simulink model "uavStepResponse"  (R2021b)
settings: configuration reference "ctrlConfigSet" (kept outside this file)
values from neighbouring files (symbols this model uses):
  TFinal = 200.0    [uavStepResponseData.sldd]
libraries: uavalgslib x1
settings Model: DataDictionary=uavStepResponseData.sldd  EnableAccessToBaseWorkspace=off  SimulationMode=accelerator  Creator=The MathWorks, Inc.  LastModifiedBy=The MathWorks, Inc.
settings ConfigSetRef: SourceName=ctrlConfigSet

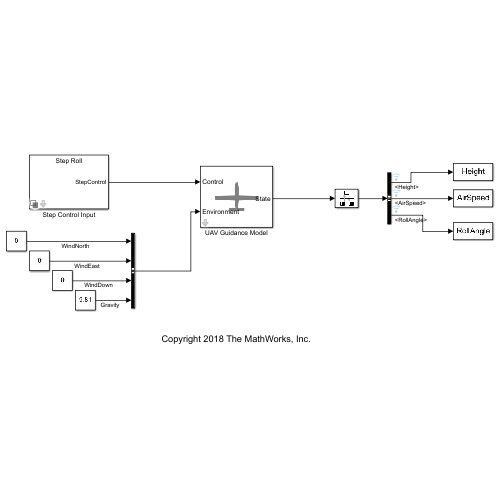
[thumbnail: Simulink's stored preview of the top-level diagram]
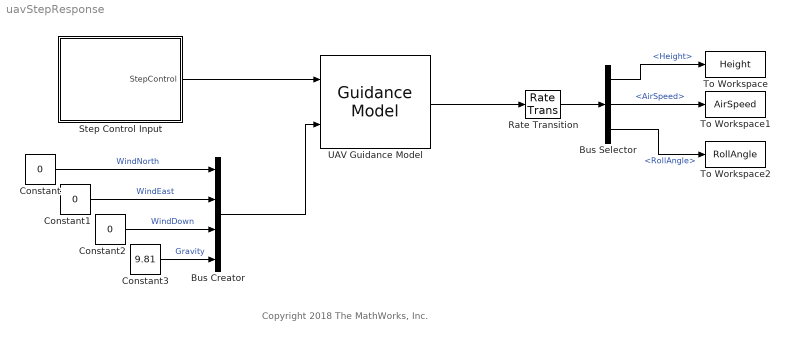
== system uavStepResponse ==
  note: Copyright 2018 The MathWorks, Inc.
  Bus Creator : BusCreator  Inputs=4  OutDataTypeStr=Bus: FixedWingEnvironmentBus  NonVirtualBus=on
  Bus Selector : BusSelector  OutputSignals=Height,AirSpeed,RollAngle
  Constant : Constant  Value=0
  Constant1 : Constant  Value=0
  Constant2 : Constant  Value=0
  Constant3 : Constant  Value=9.81
  Rate Transition : RateTransition  OutPortSampleTime=0.1
  Step Control Input : Subsystem  Variant=on  VariantControlMode=label  LabelModeActiveChoice=StepRollAngle  mask{StepControl=RollAngle Step Control}
      mask prompts: StepControl "Step control mode:"
      mask init:
      | switch StepControl
      |     case 1
      |         set_param(gcb,'LabelModeActiveChoice', 'StepHeight');
      |     case 2
      |         set_param(gcb,'LabelModeActiveChoice', 'StepAirSpeed');
      |     case 3
      |         set_param(gcb,'LabelModeActiveChoice', 'StepRollAngle');
      | end
      mask TypeOptions StepControl: Height Step Control | AirSpeed Step Control | RollAngle Step Control
  To Workspace : ToWorkspace  VariableName=Height  SaveFormat=Timeseries  SampleTime=-1
  To Workspace1 : ToWorkspace  VariableName=AirSpeed  SaveFormat=Timeseries  SampleTime=-1
  To Workspace2 : ToWorkspace  VariableName=RollAngle  SaveFormat=Timeseries  SampleTime=-1
  UAV Guidance Model : uavalgslib/Guidance Model  ModelType=FixedWingGuidance  SpecifiedDataType=double  SimulateUsing=Code generation  InitialWorldPositionMultirotor=[0; 0; 0]  InitialWorldVelocityMultirotor=[0; 0; 0]  InitialEulerZYXMultirotor=[0; 0; 0]  InitialBodyAngularRateRPYMultirotor=[0; 0; 0]  InitialThrustMultirotor=0  InitialNorthFixedWing=0  InitialEastFixedWing=0  InitialHeightFixedWing=0  InitialAirSpeedFixedWing=15  InitialHeadingAngleFixedWing=0  InitialFlightPathAngleFixedWing=0  InitialRollAngleFixedWing=0  InitialRollAngleRateFixedWing=0  PDRollMultirotor=[3402.97,116.67]  PDPitchMultirotor=[3402.97, 116.67]  PYawRateMultirotor=1950  PThrustMultirotor=3900  MassMultirotor=0.1  PHeightFixedWing=3.9  PHeadingAngleFixedWing=3.9  PFlightPathAngleFixedWing=39  PDRollFixedWing=[5.9414, 3.9]  PAirSpeedFixedWing=1  FlightPathAngleLimitsFixedWing=[-pi/6, pi/6]  StateBusName='FixedWingStateBus'  ControlBusName='FixedWingControlBus'  EnvironmentBusName='FixedWingEnvironmentBus'  DataType=double
      settings: SourceProductBaseCode=UV
  wires:
  Bus Selector/1 -> To Workspace/1  "<Height>"
  Bus Selector/2 -> To Workspace1/1  "<AirSpeed>"
  Bus Selector/3 -> To Workspace2/1  "<RollAngle>"
  Step Control Input/1(StepControl) -> UAV Guidance Model/1
  UAV Guidance Model/1 -> Rate Transition/1
  Rate Transition/1 -> Bus Selector/1
  Bus Creator/1 -> UAV Guidance Model/2
  Constant/1 -> Bus Creator/1  "WindNorth"
  Constant1/1 -> Bus Creator/2  "WindEast"
  Constant2/1 -> Bus Creator/3  "WindDown"
  Constant3/1 -> Bus Creator/4  "Gravity"

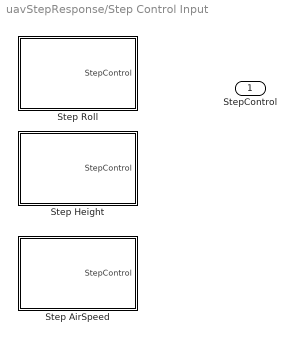
== system uavStepResponse/Step Control Input ==
  Step AirSpeed : Subsystem  VariantControl=StepAirSpeed
  Step Height : Subsystem  VariantControl=StepHeight
  Step Roll : Subsystem  VariantControl=StepRollAngle
  StepControl : Outport  VectorParamsAs1DForOutWhenUnconnected=off

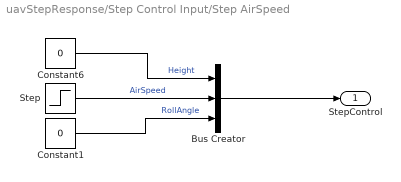
== system uavStepResponse/Step Control Input/Step AirSpeed ==
  Bus Creator : BusCreator  Inputs=3  OutDataTypeStr=Bus: FixedWingControlBus  NonVirtualBus=on
  Constant1 : Constant  Value=0
  Constant6 : Constant  Value=0
  Step : Step  Time=TFinal/2  Before=15  After=16  SampleTime=0
  StepControl : Outport  VectorParamsAs1DForOutWhenUnconnected=off
  wires:
  Constant1/1 -> Bus Creator/3  "RollAngle"
  Constant6/1 -> Bus Creator/1  "Height"
  Step/1 -> Bus Creator/2  "AirSpeed"
  Bus Creator/1 -> StepControl/1

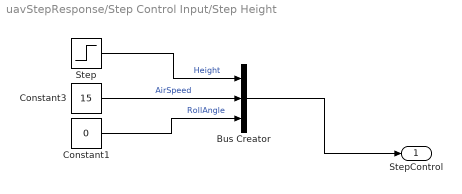
== system uavStepResponse/Step Control Input/Step Height ==
  Bus Creator : BusCreator  Inputs=3  OutDataTypeStr=Bus: FixedWingControlBus  NonVirtualBus=on
  Constant1 : Constant  Value=0
  Constant3 : Constant  Value=15
  Step : Step  Time=TFinal/2  After=5  SampleTime=0
  StepControl : Outport  VectorParamsAs1DForOutWhenUnconnected=off
  wires:
  Bus Creator/1 -> StepControl/1
  Constant3/1 -> Bus Creator/2  "AirSpeed"
  Step/1 -> Bus Creator/1  "Height"
  Constant1/1 -> Bus Creator/3  "RollAngle"

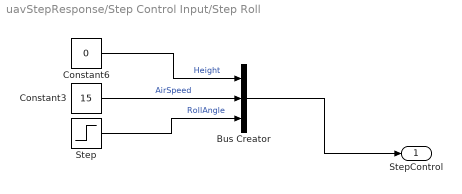
== system uavStepResponse/Step Control Input/Step Roll ==
  Bus Creator : BusCreator  Inputs=3  OutDataTypeStr=Bus: FixedWingControlBus  NonVirtualBus=on
  Constant3 : Constant  Value=15
  Constant6 : Constant  Value=0
  Step : Step  Time=TFinal/2  After=pi/6  SampleTime=0
  StepControl : Outport  VectorParamsAs1DForOutWhenUnconnected=off
  wires:
  Step/1 -> Bus Creator/3  "RollAngle"
  Constant6/1 -> Bus Creator/1  "Height"
  Constant3/1 -> Bus Creator/2  "AirSpeed"
  Bus Creator/1 -> StepControl/1
